simulink model "actuated_pendulum"  (R2026a)
settings: Solver=ode15s  StopTime=20  MaxStep=0.01  AbsTol=1e-3  EnableMultiTasking=on
values from neighbouring files (symbols this model uses):
  Ad = sys_d.A    [pendulum_script.m]    (also in run_simulator.m = M(1:2, 1:2))
  Bd = sys_d.B    [pendulum_script.m]    (also in run_simulator.m = M(1:2, 3))
  C = [1 0]    [pendulum_script.m]    (also in run_simulator.m = [1, 0])
  K = dlqr(Ad,Bd,Q,R)    [pendulum_script.m]    (also in run_simulator.m = (R + Bd' * P * Bd) \ (Bd' * P * Ad))
  L = place(Ad', C', [0.5 0.6])'    [pendulum_script.m]    (also in run_simulator.m = Delta_Ad * (Obs_mat \ [0; 1]))
  N = round(T_end / Ts)    [run_simulator.m]
  Ts = 0.02    [pendulum_script.m]    (also in run_simulator.m = 0.01)
  umax = 10    [pendulum_script.m]    (also in run_simulator.m = 2.3)
  umin = -10    [pendulum_script.m]    (also in run_simulator.m = -2.3)
  xhat0 = double([p.theta0*pi/180; p.omega0])    [pendulum_script.m]
undefined symbols (not defined in the file or in its folder): p, X, Y, Z
libraries: sm_lib x5, nesl_utility x4
settings Model: Creator=basak  LastModifiedBy=paolapinna
settings DebuggingCC: SubsystemReferenceDiagnosticForUnitTest=warning
settings SimscapeCC: SimscapeNominalValues="[{\"value\":\"1\",\"unit\":\"A\"},{\"value\":\"1\",\"unit\":\"bar\"},{\"value\":\"1\",\"unit\":\"cm^2\"},{\"value\":\"1\",\"unit\":\"cm^3/s\"},{\"value\":\"1\",\"unit\":\"kJ/kg\"},{\"value\":\"1\",\"unit\":\"kW\"},{\"value\":\"1\",\"unit\":\"l\"},{\"value\":\"1\",\"unit\":\"N\"},{\"value\":\"1\",\"unit\":\"N*m\"},{\"value\":\"1\",\"unit\":\"V\"}]"  SimscapeLogSimulationStatistics=on
settings ExplorerConfigSet: InternalSimMechanicsExplorerSettings=|
  | <ExplorerConfiguration>
  | 
  |   <canonicalview>planar_xy</canonicalview>
  | 
  |   <TilePanel>
  |     <TileInfo>
  |       <Tiles Columns="1" Count="1" Height="610" Rows="1" Width="1078">
  |         <Row Weight="1"/>
  |         <Column Weight="1"/>
  |         <Tile Height="1" Width="1" X="0" Y="0"/>
  |       </Tiles>
  |     </TileInfo>
  |     <SceneInfo>
  |       <SceneViewer>
  |         <IsThisViewStd>
  |           <IsStandardView>off</IsStandardView>
  |           <StandardViewName>Front</StandardViewName>
  |         </IsThisViewStd>
  |         <BGColor>
  |           <R>1</R>
  |           <G>1</G>
  |           <B>1</B>
  |           <A>1</A>
  |         </BGColor>
  |         <Camera>
  |           <DoPerspective>off</DoPerspective>
  |           <Position>
  |             <X>-0.14338999999999996</X>
  |             <Y>0.20478999999999997</Y>
  |             <Z>1.6177429540431678</Z>
  |           </Position>
  |           <Center>
  |             <X>-0.14338999999999996</X>
  |             <Y>0.20478999999999997</Y>
  |             <Z>0</Z>
  |           </Center>
  |           <Up>
  |             <X>0</X>
  |             <Y>1</Y>
  |             <Z>0</Z>
  |           </Up>
  |           <XLim>0.22274687273589744</XLim>
  |           <YLim>0.22274687273589744</YLim>
  |           <ViewLimDist>0.01</ViewLimDist>
  |         </Camera>
  |       </SceneViewer>
  |     </SceneInfo>
  |   </TilePanel>
  | 
  |   <MechEditorPanel>
  |     <GfxPanelCameraMap/>
  |     <Cameras/>
  |     <VideoCreator>
  |       <IncludeTiles>All</IncludeTiles>
  |       <IncludeTime>on</IncludeTime>
  |       <IncludeWorldFrame>off</IncludeWorldFrame>
  |       <PlaybackSpeedRatio>1</PlaybackSpeedRatio>
  |       <FrameRate>30</FrameRate>
  |       <FrameSize>auto</FrameSize>
  |       <VideoFormat>UncompressedAVI</VideoFormat>
  |     </VideoCreator>
  |   </MechEditorPanel>
  | 
  |   <PlaybackSettings>
  |     <PlaybackSpeedFactor>1</PlaybackSpeedFactor>
  |   </PlaybackSettings>
  | 
  | </ExplorerConfiguration>

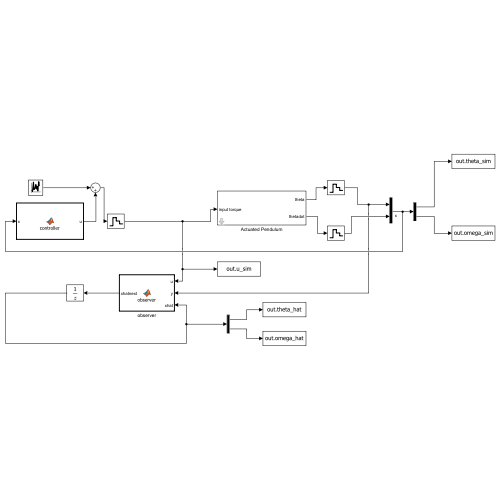
[thumbnail: Simulink's stored preview of the top-level diagram]
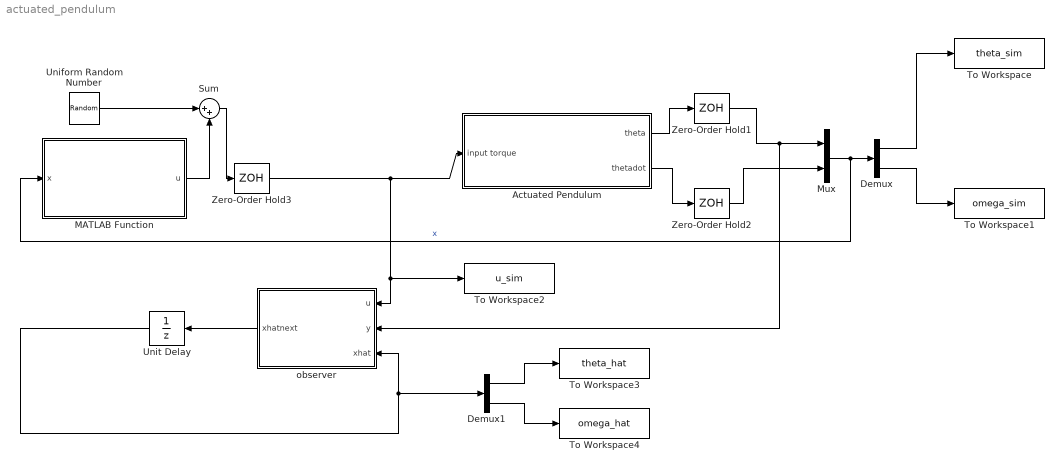
== system actuated_pendulum ==
  Actuated Pendulum : Subsystem  mask{m_p=p.m, l_p=p.l, b_p=p.b, theta0=p.theta0, thetadot0=p.omega0}
      mask prompts: m_p "Pendulum mass [kg]"; l_p "Pendulum length [m]"; b_p "Damping [N m s/rad]"; theta0 "Initial angle [deg]"; thetadot0 "Initial angular velocity [rad/s]"
  Demux : Demux  Outputs=2
  Demux1 : Demux  Outputs=2
  MATLAB Function : MATLAB Function  TreatAsAtomicUnit=on
  Mux : Mux  Inputs=2
  Sum : Sum  Inputs=|++
  To Workspace : ToWorkspace  VariableName=theta_sim  SaveFormat=Timeseries  SampleTime=-1
  To Workspace1 : ToWorkspace  VariableName=omega_sim  SaveFormat=Timeseries  SampleTime=-1
  To Workspace2 : ToWorkspace  VariableName=u_sim  SaveFormat=Timeseries  SampleTime=-1
  To Workspace3 : ToWorkspace  VariableName=theta_hat  SaveFormat=Timeseries  SampleTime=-1
  To Workspace4 : ToWorkspace  VariableName=omega_hat  SaveFormat=Timeseries  SampleTime=-1
  Uniform Random Number : UniformRandomNumber  Minimum=-0.05  Maximum=0.05  SampleTime=Ts
  Unit Delay : UnitDelay  InitialCondition=xhat0  SampleTime=Ts
  Zero-Order Hold1 : ZeroOrderHold  SampleTime=Ts
  Zero-Order Hold2 : ZeroOrderHold  SampleTime=Ts
  Zero-Order Hold3 : ZeroOrderHold  SampleTime=Ts
  observer : MATLAB Function  TreatAsAtomicUnit=on
  wires:
  Mux/1 -> MATLAB Function/1(x), Demux/1  "x"
  Demux/1 -> To Workspace/1
  Demux/2 -> To Workspace1/1
  observer/1(xhatnext) -> Unit Delay/1
  Unit Delay/1 -> observer/3(xhat), Demux1/1
  Actuated Pendulum/1(theta) -> Zero-Order Hold1/1
  Actuated Pendulum/2(thetadot) -> Zero-Order Hold2/1
  Zero-Order Hold2/1 -> Mux/2
  Demux1/1 -> To Workspace3/1
  Demux1/2 -> To Workspace4/1
  Zero-Order Hold1/1 -> observer/2(y), Mux/1
  Zero-Order Hold3/1 -> observer/1(u), To Workspace2/1, Actuated Pendulum/1(input torque)
  Uniform Random Number/1 -> Sum/1
  MATLAB Function/1(u) -> Sum/2
  Sum/1 -> Zero-Order Hold3/1

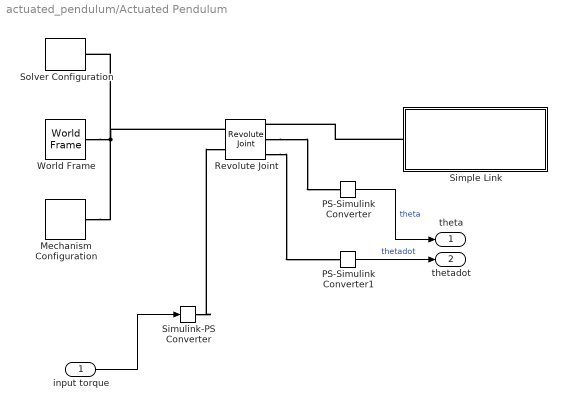
== system actuated_pendulum/Actuated Pendulum ==
  input torque : Inport
  Mechanism Configuration : sm_lib/Utilities/Mechanism Configuration  UniformGravity=Constant  GravityVector=[0 -9.81 0]  GravityVectorUnits=m/s^2  LinearizationDelta=0.001  JointModeTransitionNonlinearIterations=2
  PS-Simulink Converter : nesl_utility/PS-Simulink Converter  PhysicalDomain=network_engine_domain  SubClassName=ps_output  LeftPortType=input  RightPortType=output  PseudoPeriodic=off  Frequencies=[]  VectorFormat=inherit  Unit=inherit  AffineConversion=off
  PS-Simulink Converter1 : nesl_utility/PS-Simulink Converter  PhysicalDomain=network_engine_domain  SubClassName=ps_output  LeftPortType=input  RightPortType=output  PseudoPeriodic=off  Frequencies=[]  VectorFormat=inherit  Unit=inherit  AffineConversion=off
  Revolute Joint : sm_lib/Joints/Revolute Joint  JointMode=Normal  CompositeWrenchDir=FollowerOnBase  CompositeWrenchFrame=BaseFrame  SenseConstraintForce=off  SenseConstraintTorque=off  SenseTotalForce=off  SenseTotalTorque=off  PositionTargetSpecify=on  PositionTargetPriority=High  PositionTargetValue=theta0  PositionTargetValueUnits=deg  VelocityTargetSpecify=on  VelocityTargetPriority=High  VelocityTargetValue=thetadot0  VelocityTargetValueUnits=deg/s  EquilibriumPosition=0  EquilibriumPositionUnits=deg  SpringStiffness=0  SpringStiffnessUnits=N*m/deg  DampingCoefficient=b_p  DampingCoefficientUnits=N*m*s/rad  LowerLimitSpecify=off  LowerLimitBound=-90  LowerLimitBoundUnits=deg  LowerLimitStiffness=1e4  LowerLimitStiffnessUnits=N*m/deg  LowerLimitDamping=10  LowerLimitDampingUnits=N*m/(deg/s)  LowerLimitTransitionRegionWidth=0.1  LowerLimitTransitionRegionWidthUnits=deg  UpperLimitSpecify=off  UpperLimitBound=90  UpperLimitBoundUnits=deg  UpperLimitStiffness=1e4  UpperLimitStiffnessUnits=N*m/deg  UpperLimitDamping=10  UpperLimitDampingUnits=N*m/(deg/s)  UpperLimitTransitionRegionWidth=0.1  UpperLimitTransitionRegionWidthUnits=deg  TorqueActuationMode=InputTorque  MotionActuationMode=ComputedMotion  SensePosition=on  SenseVelocity=on  SenseAcceleration=off  SenseTorqueForce=off  SenseLowerLimitTorqueForce=off  SenseUpperLimitTorqueForce=off
  Simple Link : Subsystem  mask{L=l_p, W=0.04, H=0.04, rho=m_p, rgb=[0.25 0.40 0.70]}
      mask prompts: L "Length (m)"; W "Width (m)"; H "Thickness (m)"; rho "mass (kg)"; rgb "Color [R G B]"
  Simulink-PS Converter : nesl_utility/Simulink-PS Converter  PhysicalDomain=network_engine_domain  SubClassName=ps_input  LeftPortType=input  RightPortType=output  PseudoPeriodic=off  Frequencies=[]  NoiseDistribution=none  NoiseParameters=[]  Unit=1  AffineConversion=off  FilteringAndDerivatives=provide  SimscapeFilterOrder=1  InputFilterTimeConstant=0.001  UdotUserProvided=0
  Solver Configuration : nesl_utility/Solver Configuration  PhysicalDomain=network_engine_domain  SubClassName=solver  LeftPortType=input  RightPortType=generic  Tones=[]  Harmonics=[]  SimulateNoise=off  Profile=off  UseLocalSampling=off  EnableSwitchedLinearOptims=on  FrequencyDomain=off  UseCCode=off  RelTol=0.001  AbsTol=1e-06  MinStep=1e-09  ToWorkspace=off  RevertToSquareIcSolve=off  NumHomotopyIterations=100  PhasorMode=off  PhasorModeNumHarmonics=1  ConsistencySolver=NEWTON_XTOL_AFTER_FTOL  CanonicalOrdering=UNORDERED  OptimizeIntermediates=UNOPTIMIZED  IndexReductionMethod=DerivativeReplacement  DoDC=off  ResidualTolerance=1e-09  ConsistencyTolSource=GLOBAL  ConsistencyAbsTol=0.001  ConsistencyRelTol=0.001  ConsistencyTolFactor=0.001  UseLocalSolver=off  LocalSolverChoice=NE_BACKWARD_EULER_ADVANCER  ResolveIndetEquations=on  FunctionEvalNumThread=1  LocalSolverSampleTime=0.001  DoFixedCost=off  MaxNonlinIter=3  MaxModeIter=2  ComputeImpulses=off  ImpulseIterations=2  LinearAlgebra=Sparse  LinearAlgebraNumThread=0  EquationFormulation=NE_TIME_EF  DelaysMemoryBudget=1024  AutomaticFiltering=on  FilteringTimeConstant=0.001  PartitionStorageMethod=AS_NEEDED  PartitionMemoryBudget=1024  PartitionMethod=FAST  MultibodyUseLocalSolver=off  MultibodyLocalSolverChoice=ODE1  MultibodyLocalSolverSampleTime=0.001
  World Frame : sm_lib/Frames and Transforms/World Frame
  theta : Outport
  thetadot : Outport  Port=2
  wires:
  input torque/1 -> Simulink-PS Converter/1
  PS-Simulink Converter/1 -> theta/1  "theta"
  PS-Simulink Converter1/1 -> thetadot/1  "thetadot"
  connections:
  Simple Link/LConn1 -- Revolute Joint/RConn1
  Revolute Joint/RConn2 -- PS-Simulink Converter/LConn1
  Revolute Joint/RConn3 -- PS-Simulink Converter1/LConn1
  Simulink-PS Converter/RConn1 -- Revolute Joint/LConn2
  World Frame/RConn1 -- Revolute Joint/LConn1 -- Solver Configuration/RConn1 -- Mechanism Configuration/RConn1

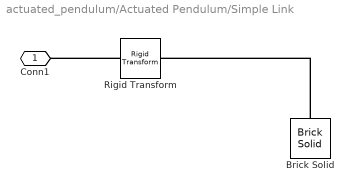
== system actuated_pendulum/Actuated Pendulum/Simple Link ==
  Brick Solid : sm_lib/Body Elements/Brick Solid  BrickDimensions=[W l_p H]  BrickDimensionsUnits=m  ExportEntireGeometry=off  InertiaType=PointMass  BasedOnType=Density  Density=rho  DensityUnits=kg/m^3  Mass=m_p  MassUnits=kg  CenterOfMass=[0 0 0]  CenterOfMassUnits=m  MomentsOfInertia=[1 1 1]  MomentsOfInertiaUnits=kg*m^2  ProductsOfInertia=[0 0 0]  ProductsOfInertiaUnits=kg*m^2  GraphicType=FromGeometry  MarkerShape=Sphere  MarkerSize=10  GraphicVisPropType=AdvancedVisualProperties  GraphicDiffuseColor=rgb  GraphicOpacity=1.0  GraphicSpecularColor=[0.5 0.5 0.5 1.0]  GraphicAmbientColor=[0.15 0.15 0.15 1.0]  GraphicEmissiveColor=[0.0 0.0 0.0 1.0]  GraphicShininess=75  DoExposeReferenceFrame=on  SerializedFrames=<Frames/>
  Rigid Transform : sm_lib/Frames and Transforms/Rigid Transform  RotationMethod=None  FollAlignAxisA=+X  BaseAlignAxisA=+Y  FollAlignAxisB=+Y  BaseAlignAxisB=+Z  RotationStandardAxis=+Z  RotationAngle=0.0  RotationAngleUnits=deg  RotationArbitraryAxis=[0 0 1]  RotationSequenceAxes=FollowerAxes  RotationSequence=XYX  RotationSequenceAngles=[0 0 0]  RotationSequenceAnglesUnits=deg  RotationMatrix=[1 0 0; 0 1 0; 0 0 1]  Quaternion=[1 0 0 0]  TranslationMethod=Cartesian  TranslationCartesianOffset=[0 -L/2 0]  TranslationCartesianOffsetUnits=m  TranslationStandardAxis=+Y  TranslationStandardOffset=L/2  TranslationStandardOffsetUnits=m  TranslationROffset=0  TranslationROffsetUnits=m  TranslationThetaOffset=0  TranslationThetaOffsetUnits=deg  TranslationZOffset=0  TranslationZOffsetUnits=m
  Conn1 : PMIOPort  Side=Left
  connections:
  Rigid Transform/RConn1 -- Conn1/RConn1
  Brick Solid/RConn1 -- Rigid Transform/LConn1

== matlab function actuated_pendulum/observer ==
  data: u input; y input; xhat input; Ad parameter; Bd parameter; L parameter; C parameter; xhatnext output

function xhatnext = observer(u, y, xhat, Ad, Bd, L, C)

    xhatnext = Ad*xhat + Bd*u + L*(y - C*xhat);

end

== matlab function actuated_pendulum/MATLAB Function ==
  data: x input; u output; K parameter; umin parameter; umax parameter
function u = controller(x, K, umin, umax)

% LQR control law
u = -K*x;

% Actuator saturation
u = min(max(u, umin), umax);

end
